simulink model "inverter_real_unidad"  (R2026b)
settings: Solver=VariableStepAuto
values from neighbouring files (symbols this model uses):
  wn_V = 6000    [coeficientes.m]
  zeta_V = 1    [coeficientes.m]
settings Model: Creator=lamun  LastModifiedBy=lamun

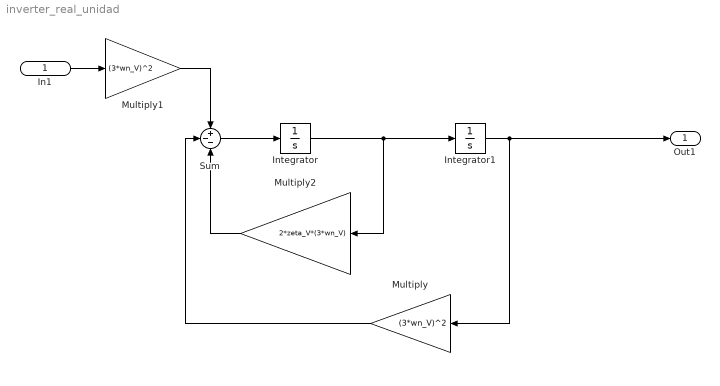
== system inverter_real_unidad ==
  In1 : Inport
  Integrator : Integrator
  Integrator1 : Integrator
  Multiply : Gain  Gain=(3*wn_V)^2
  Multiply1 : Gain  Gain=(3*wn_V)^2
  Multiply2 : Gain  Gain=2*zeta_V*(3*wn_V)
  Sum : Sum  Inputs=+--
  Out1 : Outport
  wires:
  Sum/1 -> Integrator/1
  Integrator1/1 -> Multiply/1, Out1/1
  Multiply/1 -> Sum/2
  Integrator/1 -> Multiply2/1, Integrator1/1
  Multiply2/1 -> Sum/3
  Multiply1/1 -> Sum/1
  In1/1 -> Multiply1/1
